simulink model "boucle_tangage"  (R2025b)
settings: Solver=FixedStepAuto  StartTime=0.0  StopTime=5  FixedStep=Ts  RelTol=1e-3
values from neighbouring files (symbols this model uses):
  Kd = 0.015    [generer_bdd_x_theta.m]
  Kdpsi = 0.03    [generer_bdd_x_theta.m]
  Kp = 0.02    [generer_bdd_x_theta.m]
  Kpsi = 0.04    [generer_bdd_x_theta.m]
  Ts = 0.05    [generer_bdd_x_theta.m]
  u0 = 0.386    [generer_bdd_x_theta.m]
undefined symbols (not defined in the file or in its folder): DiscIntNeverNeededParam
settings Model: Creator=nicol  LastModifiedBy=nicol
settings SolverCC: AlgebraicLoopSolver=TrustRegion
settings DebuggingCC: UnconnectedInputMsg=warning  UnconnectedOutputMsg=warning  UnconnectedLineMsg=warning
settings ModelReferenceCC: EnableRefExpFcnMdlSchedulingChecks=on
settings RTWCC: GPUComputeCapability=3.5

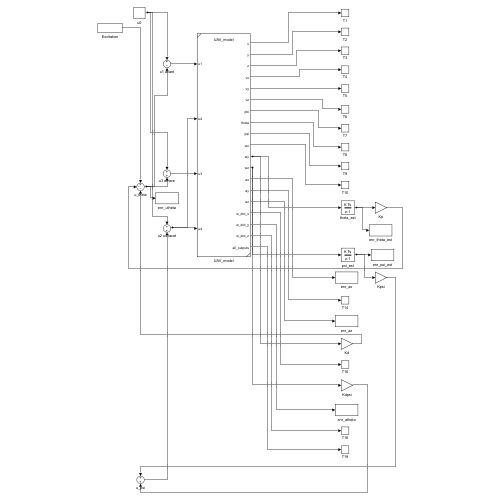
[thumbnail: Simulink's stored preview of the top-level diagram]
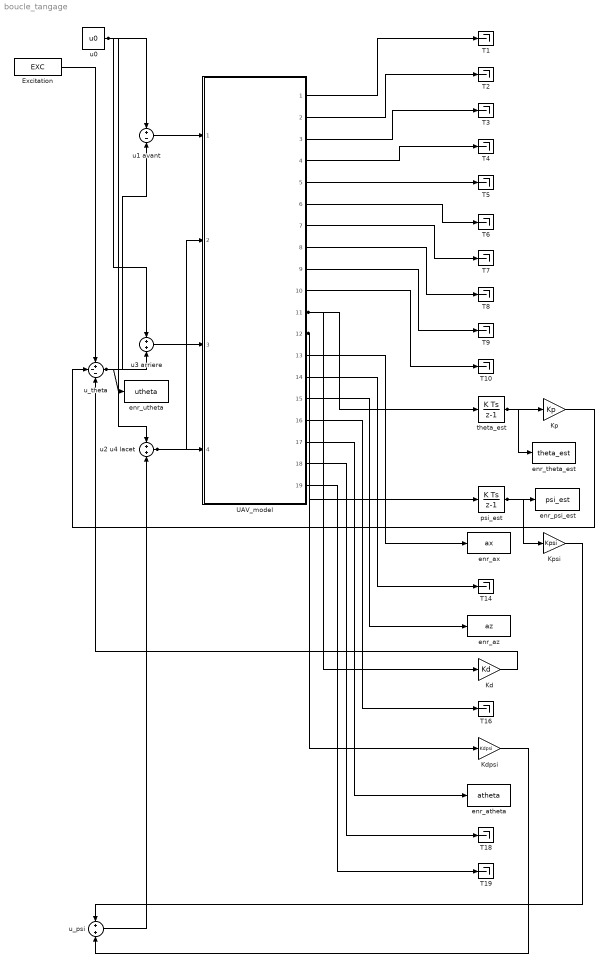
== system boucle_tangage ==
  Excitation : FromWorkspace  VariableName=EXC  SampleTime=Ts  Interpolate=off  OutputAfterFinalValue=Holding final value
  Kd : Gain  Gain=Kd
  Kdpsi : Gain  Gain=Kdpsi
  Kp : Gain  Gain=Kp
  Kpsi : Gain  Gain=Kpsi
  T{1..10,14,16,18..19} (14 alike) : Terminator
  UAV_model : Subsystem  ReferencedSubsystem=UAV_model
  enr_atheta : ToWorkspace  VariableName=atheta  SampleTime=Ts
  enr_ax : ToWorkspace  VariableName=ax  SampleTime=Ts
  enr_az : ToWorkspace  VariableName=az  SampleTime=Ts
  enr_psi_est : ToWorkspace  VariableName=psi_est  SampleTime=Ts
  enr_theta_est : ToWorkspace  VariableName=theta_est  SampleTime=Ts
  enr_utheta : ToWorkspace  VariableName=utheta  SampleTime=Ts
  psi_est : DiscreteIntegrator  gainval=1  SampleTime=Ts  ICPrevOutput=DiscIntNeverNeededParam  ICPrevScaledInput=DiscIntNeverNeededParam
  theta_est : DiscreteIntegrator  gainval=1  SampleTime=Ts  ICPrevOutput=DiscIntNeverNeededParam  ICPrevScaledInput=DiscIntNeverNeededParam
  u0 : Constant  Value=u0
  u1 avant : Sum  Inputs=+-
  u2 u4 lacet : Sum
  u3 arriere : Sum
  u_psi : Sum
  u_theta : Sum  Inputs=+--
  wires:
  UAV_model/17 -> enr_atheta/1
  Excitation/1 -> u_theta/1
  UAV_model/1 -> T1/1
  u2 u4 lacet/1 -> UAV_model/2, UAV_model/4
  psi_est/1 -> Kpsi/1, enr_psi_est/1
  theta_est/1 -> enr_theta_est/1, Kp/1
  u3 arriere/1 -> UAV_model/3
  u1 avant/1 -> UAV_model/1
  u_psi/1 -> u2 u4 lacet/2
  Kp/1 -> u_theta/2
  u0/1 -> u3 arriere/1, u2 u4 lacet/1, u1 avant/1
  Kpsi/1 -> u_psi/1
  u_theta/1 -> u3 arriere/2, enr_utheta/1, u1 avant/2
  UAV_model/18 -> T18/1
  UAV_model/2 -> T2/1
  UAV_model/19 -> T19/1
  UAV_model/3 -> T3/1
  UAV_model/4 -> T4/1
  UAV_model/5 -> T5/1
  UAV_model/6 -> T6/1
  UAV_model/7 -> T7/1
  UAV_model/8 -> T8/1
  UAV_model/9 -> T9/1
  UAV_model/10 -> T10/1
  UAV_model/11 -> theta_est/1, Kd/1
  UAV_model/12 -> psi_est/1, Kdpsi/1
  UAV_model/13 -> enr_ax/1
  UAV_model/14 -> T14/1
  UAV_model/15 -> enr_az/1
  UAV_model/16 -> T16/1
  Kd/1 -> u_theta/3
  Kdpsi/1 -> u_psi/2
